simulink library "lib_SecCtrl_MatricesDelayLim"  (R2026a)
settings: Solver=VariableStepAuto
undefined symbols (not defined in the file): A_f_sc, A_P_sc, A_Q_sc, A_v_sc, buses_lf, costs, delayM, Qs_lf, sec_control_structure
libraries: simulink x7, sl_discontinuities x2
settings Model: Creator=atomas  LastModifiedBy=atomas

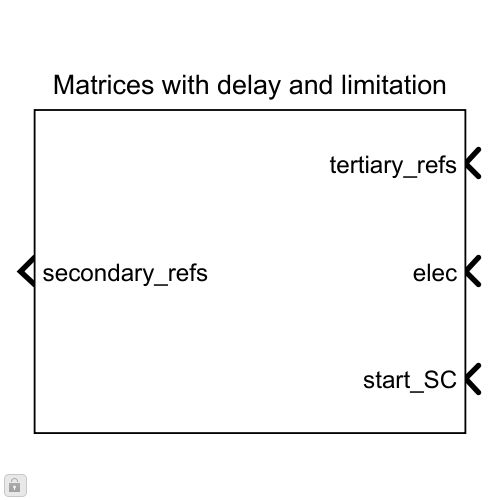
[thumbnail: Simulink's stored preview of the top-level diagram]
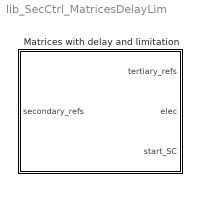
== system lib_SecCtrl_MatricesDelayLim ==
  Matrices with delay and limitation : Subsystem  VariantControl=Matrices with delay and limitation

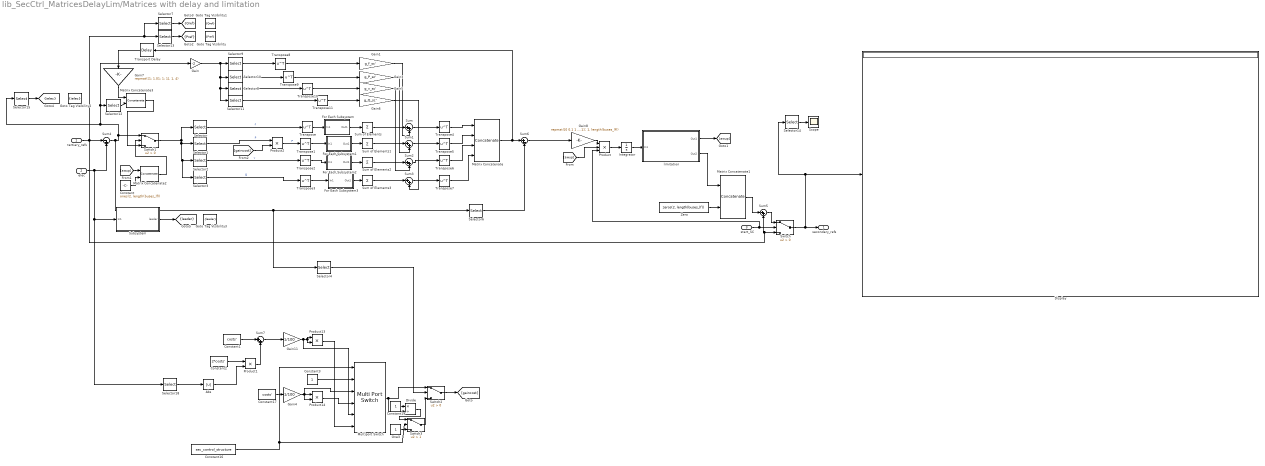
== system lib_SecCtrl_MatricesDelayLim/Matrices with delay and limitation ==
  tertiary_refs : Inport
  elec : Inport  Port=2
  start_SC : Inport  Port=3
  Abs : Abs  SaturateOnIntegerOverflow=off
  Constant : Constant  Value=ones(2, length(buses_lf))  VectorParams1D=off
  Constant1 : Constant  Value=costs'  VectorParams1D=off
  Constant16 : Constant  Value=sec_control_structure
  Constant17 : Constant  Value=costs'  VectorParams1D=off
  Constant19 : Constant  VectorParams1D=off
  Constant2 : Constant  Value=2*costs'  VectorParams1D=off
  Constant3 : Constant
  Display : Display
  Divide : Product  Inputs=*/
  For Each Subsystem : Subsystem  TreatAsAtomicUnit=on  mask{delayM=delayM, A_f_sc=A_f_sc}
  For Each Subsystem1 : Subsystem  TreatAsAtomicUnit=on  mask{delayM=delayM, A_P_sc=A_P_sc}
  For Each Subsystem2 : Subsystem  TreatAsAtomicUnit=on  mask{delayM=delayM, A_v_sc=A_v_sc}
  For Each Subsystem3 : Subsystem  TreatAsAtomicUnit=on  mask{delayM=delayM, A_Q_sc=A_Q_sc}
  Gain : Gain  Gain=-2
  Gain1 : Gain  Gain=g_f_sc'
  Gain11 : Gain  Gain=1/100
  Gain3 : Gain  Gain=g_P_sc'
  Gain4 : Gain  Gain=1/100
  Gain5 : Gain  Gain=g_v_sc'
  Gain6 : Gain  Gain=g_Q_sc'
  Gain7 : Gain  Gain=repmat([1; 1.01; 1; 1], 1, 4)
  Gain8 : Gain  Gain=repmat([0 0.1 1 0.1]', 1, length(buses_lf))
  Goto Tag Visibility : GotoTagVisibility  GotoTag=Pref
  Goto Tag Visibility1 : GotoTagVisibility  GotoTag=Qref
  Goto Tag Visibility2 : GotoTagVisibility  GotoTag=ielec
  Goto Tag Visibility3 : GotoTagVisibility  GotoTag=leader
  Integrator : Integrator
  Matrix Concatenate : Concatenate  NumInputs=4  Mode=Multidimensional array
  Matrix Concatenate1 : Concatenate  Mode=Multidimensional array
  Matrix Concatenate2 : Concatenate  Mode=Multidimensional array
  Matrix Concatenate3 : Concatenate  Mode=Multidimensional array
  Multiport Switch : MultiPortSwitch  Inputs=5  SaturateOnIntegerOverflow=off  InputSameDT=off
  One3 : Constant  OutDataTypeStr=Inherit: Inherit via back propagation
  Product : Product  Inputs=3
  Product{1..2,13..14} (4 alike) : Product
  Scope : Scope
      settings: ActiveDisplayYMinimum=0.00424  ActiveDisplayYMaximum=0.00539
  Selector : Selector  NumberOfDimensions=2  InputPortWidth=3  IndexOptions=Index vector (dialog),Select all  Indices=1,1  OutputSizes=1,1
  Selector{1,4,10,13,18} (5 alike) : Selector  NumberOfDimensions=2  InputPortWidth=3  IndexOptions=Index vector (dialog),Select all  Indices=2,1  OutputSizes=1,1
  Selector11 : Selector  NumberOfDimensions=2  InputPortWidth=3  IndexOptions=Index vector (dialog),Select all  Indices=4,1  OutputSizes=1,1
  Selector12 : Selector  NumberOfDimensions=2  InputPortWidth=3  IndexOptions=Index vector (dialog),Select all  Indices=5:6,1  OutputSizes=1,1
  Selector14 : Selector  NumberOfDimensions=2  InputPortWidth=3  IndexOptions=Index vector (dialog),Index vector (dialog)  Indices=2,1  OutputSizes=1,1
  Selector15 : Selector  NumberOfDimensions=2  InputPortWidth=3  IndexOptions=Index vector (dialog),Select all  Indices=1:4,1  OutputSizes=1,1
  Selector2 : Selector  NumberOfDimensions=2  InputPortWidth=3  IndexOptions=Index vector (dialog),Select all  Indices=3,1  OutputSizes=1,1
  Selector3 : Selector  NumberOfDimensions=2  InputPortWidth=3  IndexOptions=Index vector (dialog),Select all  Indices=4,1  OutputSizes=1,1
  Selector6 : Selector  NumberOfDimensions=2  InputPortWidth=3  IndexOptions=Index vector (dialog),Select all  Indices=1:4,1  OutputSizes=1,1
  Selector7 : Selector  NumberOfDimensions=2  InputPortWidth=3  IndexOptions=Index vector (dialog),Select all  Indices=4,1  OutputSizes=1,1
  Selector8 : Selector  NumberOfDimensions=2  InputPortWidth=3  IndexOptions=Index vector (dialog),Select all  Indices=3,1  OutputSizes=1,1
  Selector9 : Selector  NumberOfDimensions=2  InputPortWidth=3  IndexOptions=Index vector (dialog),Select all  Indices=1,1  OutputSizes=1,1
  Subsystem : Subsystem
  Sum{,1..3,5,7} (6 alike) : Sum  Inputs=|++
  Sum of Elements{,1..3} (4 alike) : Sum  Inputs=+  CollapseMode=Specified dimension  CollapseDim=2
  Sum4 : Sum  Inputs=|-+
  Sum6 : Sum  Inputs=|+-
  Switch : Switch  Criteria=u2 > Threshold  SaturateOnIntegerOverflow=off  InputSameDT=off
  Switch1 : Switch  Criteria=u2 > Threshold  SaturateOnIntegerOverflow=off  InputSameDT=off
  Switch2 : Switch  Criteria=u2 > Threshold  SaturateOnIntegerOverflow=off  InputSameDT=off
  Switch3 : Switch  Criteria=u2 > Threshold  Threshold=1  SaturateOnIntegerOverflow=off  InputSameDT=off
  Transport Delay : TransportDelay  DelayTime=1e-9
  Transpose{,1..11} (12 alike) : Math  Operator=transpose
  Zero : Constant  Value=zeros(2, length(buses_lf))  VectorParams1D=off  OutDataTypeStr=Inherit: Inherit via back propagation
  limitation : Subsystem
  secondary_refs : Outport
  tag scope: Pref=scoped, Qref=scoped, ielec=scoped, leader=scoped
  wires:
  Abs/1 -> Product1/2
  Gain7/1 -> Matrix Concatenate3/1
  Matrix Concatenate3/1 -> Switch1/3
  Selector1/1 -> Product2/1  "P"
  Constant17/1 -> Gain4/1
  Constant19/1 -> Divide/1
  Constant2/1 -> Product1/1
  Product14/1 -> Multiport Switch/4
  Constant3/1 -> Multiport Switch/2
  Switch2/1 -> [gaincost]
  Switch3/1 -> Switch2/3
  Divide/1 -> Switch3/1
  Product13/1 -> Multiport Switch/6
  Product1/1 -> Sum7/2
  Selector18/1 -> Abs/1
  Multiport Switch/1 -> Switch2/1, Divide/2
  Selector4/1 -> Switch2/2
  [gaincost] -> Product2/2
  Constant16/1 -> Multiport Switch/1, Switch3/2
  Constant1/1 -> Sum7/1
  One3/1 -> Switch3/3
  Gain11/1 -> Product13/1, Product13/2, Multiport Switch/5
  Gain4/1 -> Product14/1, Product14/2, Multiport Switch/3
  Sum7/1 -> Gain11/1
  elec/1 -> Sum4/2, Subsystem/1(In1), Selector18/1
  [awup] -> Product/2
  Product/1 -> Integrator/1
  Integrator/1 -> limitation/1(In1)
  Sum6/1 -> Gain8/1
  Zero/1 -> Matrix Concatenate1/2
  tertiary_refs/1 -> Sum4/1, Selector13/1, Selector7/1, Switch/3, Sum5/2
  Selector15/1 -> [ielec]
  Subsystem/1(leader) -> [leader]
  Selector14/1 -> Scope/1
  Transport Delay/1 -> Gain7/1
  Selector12/1 -> Matrix Concatenate3/2
  Sum4/1 -> Selector6/1, Selector4/1, Selector12/1, Gain/1, Selector15/1, Switch1/1
  Constant/1 -> Matrix Concatenate2/2
  [awup] -> Matrix Concatenate2/1
  Matrix Concatenate2/1 -> Switch1/2
  Gain8/1 -> Product/1
  limitation/2(Out2) -> Matrix Concatenate1/1
  limitation/1(Out1) -> [awup]
  Selector7/1 -> [Qref]
  Selector13/1 -> [Pref]
  Gain/1 -> Selector9/1, Selector10/1, Selector8/1, Selector11/1
  Transpose11/1 -> Gain6/1
  Transpose10/1 -> Gain5/1
  Transpose9/1 -> Gain3/1
  Transpose8/1 -> Gain1/1
  start_SC/1 -> Switch/2, Product/3
  Selector6/1 -> Sum6/2
  Matrix Concatenate/1 -> Sum6/1, Transport Delay/1
  Selector9/1 -> Transpose8/1
  Switch1/1 -> Selector/1, Selector1/1, Selector3/1, Selector2/1
  Selector11/1 -> Transpose11/1
  Selector8/1 -> Transpose10/1
  Selector10/1 -> Transpose9/1
  Sum5/1 -> Switch/1
  Matrix Concatenate1/1 -> Sum5/1
  Transpose5/1 -> Matrix Concatenate/2
  Switch/1 -> secondary_refs/1, Display/1, Selector14/1
  For Each Subsystem3/1(Out1) -> Sum of Elements3/1
  For Each Subsystem2/1(Out1) -> Sum of Elements2/1
  For Each Subsystem1/1(Out1) -> Sum of Elements1/1
  For Each Subsystem/1(Out1) -> Sum of Elements/1
  Sum of Elements/1 -> Sum/1
  Transpose7/1 -> Matrix Concatenate/4
  Transpose6/1 -> Matrix Concatenate/3
  Transpose4/1 -> Matrix Concatenate/1
  Transpose3/1 -> For Each Subsystem3/1(In1)
  Transpose2/1 -> For Each Subsystem2/1(In1)
  Transpose1/1 -> For Each Subsystem1/1(In1)
  Transpose/1 -> For Each Subsystem/1(In1)
  Sum of Elements3/1 -> Sum3/1
  Sum3/1 -> Transpose7/1
  Sum2/1 -> Transpose6/1
  Gain6/1 -> Sum3/2
  Gain5/1 -> Sum2/2
  Sum of Elements2/1 -> Sum2/1
  Sum1/1 -> Transpose5/1
  Gain3/1 -> Sum1/2
  Sum of Elements1/1 -> Sum1/1
  Gain1/1 -> Sum/2
  Sum/1 -> Transpose4/1
  Selector2/1 -> Transpose2/1  "v"
  Product2/1 -> Transpose1/1  "P"
  Selector/1 -> Transpose/1  "f"
  Selector3/1 -> Transpose3/1  "Q"

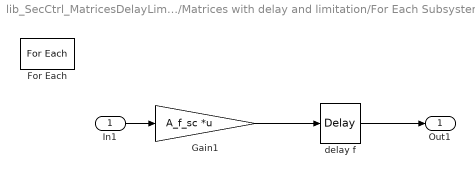
== system lib_SecCtrl_MatricesDelayLim/Matrices with delay and limitation/For Each Subsystem ==
  In1 : Inport  Partition=on  PartitionDimension=1  PartitionWidth=1  PartitionOffset=0
  For Each : ForEach  DisableCoverage=on  IterateSubsysMaskParameter=on,on  SubsysMaskParameterIterationDimension=2,2
  Gain1 : Gain  Gain=A_f_sc  Multiplication=Matrix(K*u)
  delay f : TransportDelay  DelayTime=delayM  PadeOrder=3
  Out1 : Outport  ConcatenationDimension=2
  wires:
  delay f/1 -> Out1/1
  Gain1/1 -> delay f/1
  In1/1 -> Gain1/1

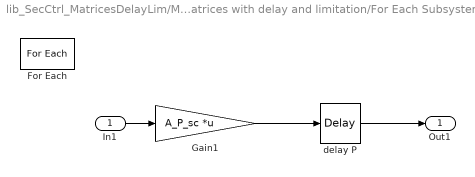
== system lib_SecCtrl_MatricesDelayLim/Matrices with delay and limitation/For Each Subsystem1 ==
  In1 : Inport  Partition=on  PartitionDimension=1  PartitionWidth=1  PartitionOffset=0
  For Each : ForEach  DisableCoverage=on  IterateSubsysMaskParameter=on,on  SubsysMaskParameterIterationDimension=2,2
  Gain1 : Gain  Gain=A_P_sc  Multiplication=Matrix(K*u)
  delay P : TransportDelay  DelayTime=delayM  PadeOrder=3
  Out1 : Outport  ConcatenationDimension=2
  wires:
  In1/1 -> Gain1/1
  Gain1/1 -> delay P/1
  delay P/1 -> Out1/1

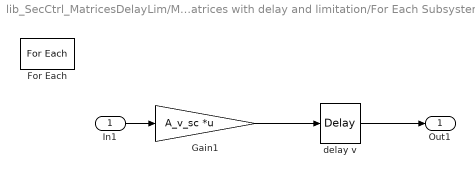
== system lib_SecCtrl_MatricesDelayLim/Matrices with delay and limitation/For Each Subsystem2 ==
  In1 : Inport  Partition=on  PartitionDimension=1  PartitionWidth=1  PartitionOffset=0
  For Each : ForEach  DisableCoverage=on  IterateSubsysMaskParameter=on,on  SubsysMaskParameterIterationDimension=2,2
  Gain1 : Gain  Gain=A_v_sc  Multiplication=Matrix(K*u)
  delay v : TransportDelay  DelayTime=delayM  PadeOrder=3
  Out1 : Outport  ConcatenationDimension=2
  wires:
  delay v/1 -> Out1/1
  Gain1/1 -> delay v/1
  In1/1 -> Gain1/1

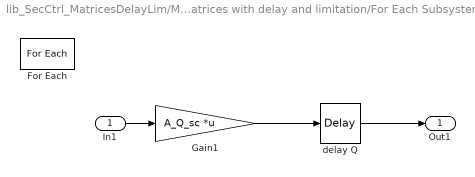
== system lib_SecCtrl_MatricesDelayLim/Matrices with delay and limitation/For Each Subsystem3 ==
  In1 : Inport  Partition=on  PartitionDimension=1  PartitionWidth=1  PartitionOffset=0
  For Each : ForEach  DisableCoverage=on  IterateSubsysMaskParameter=on,on  SubsysMaskParameterIterationDimension=2,2
  Gain1 : Gain  Gain=A_Q_sc  Multiplication=Matrix(K*u)
  delay Q : TransportDelay  DelayTime=delayM  PadeOrder=3
  Out1 : Outport  ConcatenationDimension=2
  wires:
  In1/1 -> Gain1/1
  Gain1/1 -> delay Q/1
  delay Q/1 -> Out1/1

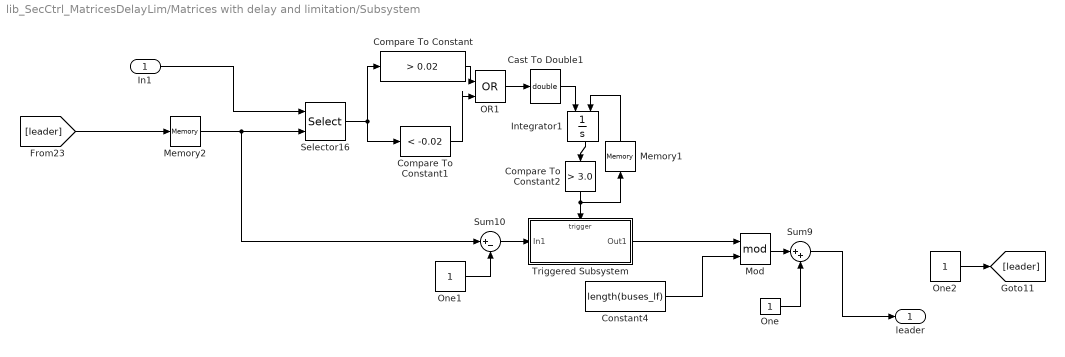
== system lib_SecCtrl_MatricesDelayLim/Matrices with delay and limitation/Subsystem ==
  In1 : Inport
  Cast To Double1 : DataTypeConversion  OutDataTypeStr=double  SaturateOnIntegerOverflow=off  RndMeth=Floor
  Compare To Constant : simulink/Logic and Bit Operations/Compare To Constant  relop=>  const=0.02  OutDataTypeStr=boolean
  Compare To Constant1 : simulink/Logic and Bit Operations/Compare To Constant  relop=<  const=-0.02  OutDataTypeStr=boolean
  Compare To Constant2 : simulink/Logic and Bit Operations/Compare To Constant  relop=>  const=3.0  OutDataTypeStr=boolean
  Constant4 : Constant  Value=length(buses_lf)
  Integrator1 : Integrator  ExternalReset=rising
  Memory1 : Memory
  Memory2 : Memory  InitialCondition=1
  Mod : Math  Operator=mod
  OR1 : Logic  Operator=OR  IconShape=distinctive  AllPortsSameDT=off  OutDataTypeStr=boolean
  One : Constant  OutDataTypeStr=Inherit: Inherit via back propagation
  One1 : Constant  OutDataTypeStr=Inherit: Inherit via back propagation
  One2 : Constant  OutDataTypeStr=Inherit: Inherit via back propagation
  Selector16 : Selector  NumberOfDimensions=2  InputPortWidth=length(buses_lf)  IndexOptions=Index vector (dialog),Index vector (port)  Indices=2,1  OutputSizes=1,1
  Sum10 : Sum  Inputs=|+-
  Sum9 : Sum  Inputs=|++
  Triggered Subsystem : Subsystem  TreatAsAtomicUnit=on
  leader : Outport
  wires:
  One2/1 -> [leader]
  Triggered Subsystem/1(Out1) -> Mod/1
  Memory1/1 -> Integrator1/2
  Sum9/1 -> leader/1
  One1/1 -> Sum10/2
  Constant4/1 -> Mod/2
  Selector16/1 -> Compare To Constant/1, Compare To Constant1/1
  Mod/1 -> Sum9/1
  In1/1 -> Selector16/1
  Sum10/1 -> Triggered Subsystem/1(In1)
  Memory2/1 -> Selector16/2, Sum10/1
  One/1 -> Sum9/2
  Compare To Constant1/1 -> OR1/2
  Cast To Double1/1 -> Integrator1/1
  Integrator1/1 -> Compare To Constant2/1
  OR1/1 -> Cast To Double1/1
  Compare To Constant2/1 -> Triggered Subsystem/Trigger, Memory1/1
  [leader] -> Memory2/1
  Compare To Constant/1 -> OR1/1

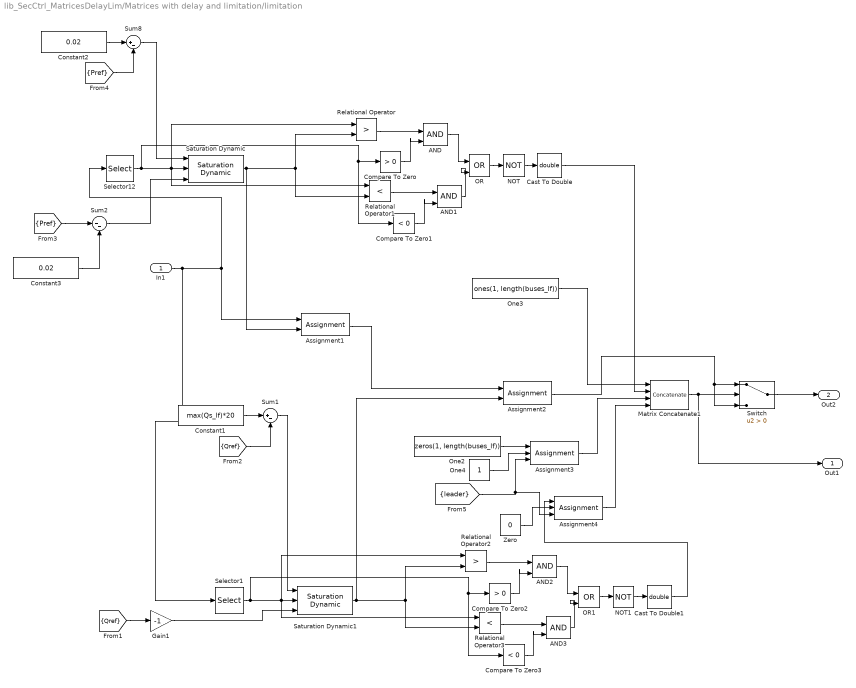
== system lib_SecCtrl_MatricesDelayLim/Matrices with delay and limitation/limitation ==
  In1 : Inport
  AND{,1..3} (4 alike) : Logic  IconShape=distinctive  AllPortsSameDT=off  OutDataTypeStr=boolean
  Assignment1 : Assignment  NumberOfDimensions=2  DiagnosticForDimensions=Warning  IndexOptions=Index vector (dialog),Assign all  Indices=2,1  OutputSizes=1,1
  Assignment2 : Assignment  NumberOfDimensions=2  DiagnosticForDimensions=Warning  IndexOptions=Index vector (dialog),Assign all  Indices=4,1  OutputSizes=1,1
  Assignment3 : Assignment  DiagnosticForDimensions=Warning  IndexOptions=Index vector (port)  Indices=4  OutputSizes=1
  Assignment4 : Assignment  DiagnosticForDimensions=Warning  IndexOptions=Index vector (port)  Indices=4  OutputSizes=1
  Cast To Double : DataTypeConversion  OutDataTypeStr=double  SaturateOnIntegerOverflow=off  RndMeth=Floor
  Cast To Double1 : DataTypeConversion  OutDataTypeStr=double  SaturateOnIntegerOverflow=off  RndMeth=Floor
  Compare To Zero : simulink/Logic and Bit Operations/Compare To Zero  relop=>  OutDataTypeStr=boolean
  Compare To Zero1 : simulink/Logic and Bit Operations/Compare To Zero  relop=<  OutDataTypeStr=boolean
  Compare To Zero2 : simulink/Logic and Bit Operations/Compare To Zero  relop=>  OutDataTypeStr=boolean
  Compare To Zero3 : simulink/Logic and Bit Operations/Compare To Zero  relop=<  OutDataTypeStr=boolean
  Constant1 : Constant  Value=max(Qs_lf)*20  VectorParams1D=off
  Constant2 : Constant  Value=0.02  VectorParams1D=off
  Constant3 : Constant  Value=0.02  VectorParams1D=off
  Gain1 : Gain  Gain=-1
  Matrix Concatenate1 : Concatenate  NumInputs=4  Mode=Multidimensional array
  NOT : Logic  Operator=NOT  IconShape=distinctive  AllPortsSameDT=off  OutDataTypeStr=boolean
  NOT1 : Logic  Operator=NOT  IconShape=distinctive  AllPortsSameDT=off  OutDataTypeStr=boolean
  OR : Logic  Operator=OR  IconShape=distinctive  AllPortsSameDT=off  OutDataTypeStr=boolean
  OR1 : Logic  Operator=OR  IconShape=distinctive  AllPortsSameDT=off  OutDataTypeStr=boolean
  One2 : Constant  Value=zeros(1, length(buses_lf))  VectorParams1D=off  OutDataTypeStr=Inherit: Inherit via back propagation
  One3 : Constant  Value=ones(1, length(buses_lf))  VectorParams1D=off  OutDataTypeStr=Inherit: Inherit via back propagation
  One4 : Constant  OutDataTypeStr=Inherit: Inherit via back propagation
  Relational Operator : RelationalOperator  Operator=>  OutDataTypeStr=boolean  RndMeth=Simplest  InputSameDT=off
  Relational Operator1 : RelationalOperator  Operator=<  OutDataTypeStr=boolean  RndMeth=Simplest  InputSameDT=off
  Relational Operator2 : RelationalOperator  Operator=>  OutDataTypeStr=boolean  RndMeth=Simplest  InputSameDT=off
  Relational Operator3 : RelationalOperator  Operator=<  OutDataTypeStr=boolean  RndMeth=Simplest  InputSameDT=off
  Saturation Dynamic : sl_discontinuities/Saturation Dynamic  OutMin=[]  OutMax=[]  OutDataTypeStr=Inherit: Same as second input  OutDataType=fixdt(1, 16)  OutScaling=2^-10  DoSatur=off
  Saturation Dynamic1 : sl_discontinuities/Saturation Dynamic  OutMin=[]  OutMax=[]  OutDataTypeStr=Inherit: Same as second input  OutDataType=fixdt(1, 16)  OutScaling=2^-10  DoSatur=off
  Selector1 : Selector  NumberOfDimensions=2  InputPortWidth=3  IndexOptions=Index vector (dialog),Select all  Indices=4,1  OutputSizes=1,1
  Selector12 : Selector  NumberOfDimensions=2  InputPortWidth=3  IndexOptions=Index vector (dialog),Select all  Indices=2,1  OutputSizes=1,1
  Sum1 : Sum  Inputs=|+-
  Sum2 : Sum  Inputs=|--
  Sum8 : Sum  Inputs=|+-
  Switch : Switch  Criteria=u2 > Threshold  SaturateOnIntegerOverflow=off  InputSameDT=off
  Zero : Constant  Value=0  OutDataTypeStr=Inherit: Inherit via back propagation
  Out1 : Outport
  Out2 : Outport  Port=2
  wires:
  Constant3/1 -> Sum2/2
  [Pref] -> Sum2/1
  Zero/1 -> Assignment4/2
  Assignment4/1 -> Matrix Concatenate1/4
  One4/1 -> Assignment3/2
  One2/1 -> Assignment3/1
  [leader] -> Assignment3/3, Assignment4/3
  Assignment3/1 -> Matrix Concatenate1/3
  One3/1 -> Matrix Concatenate1/1
  Switch/1 -> Out2/1
  Assignment2/1 -> Switch/1, Switch/3
  Matrix Concatenate1/1 -> Switch/2, Out1/1
  Compare To Zero2/1 -> AND2/2
  Cast To Double1/1 -> Assignment4/1
  In1/1 -> Assignment1/1, Selector12/1, Selector1/1
  [Qref] -> Gain1/1
  Compare To Zero3/1 -> AND3/2
  Sum1/1 -> Saturation Dynamic1/1
  AND2/1 -> OR1/1
  Relational Operator3/1 -> AND3/1
  Selector1/1 -> Compare To Zero2/1, Compare To Zero3/1, Saturation Dynamic1/2, Relational Operator2/1, Relational Operator3/1
  OR1/1 -> NOT1/1
  Gain1/1 -> Saturation Dynamic1/3
  AND3/1 -> OR1/2
  Relational Operator2/1 -> AND2/1
  [Qref] -> Sum1/2
  NOT1/1 -> Cast To Double1/1
  Constant1/1 -> Sum1/1
  Saturation Dynamic1/1 -> Relational Operator2/2, Relational Operator3/2, Assignment2/2
  Assignment1/1 -> Assignment2/1
  Cast To Double/1 -> Matrix Concatenate1/2
  NOT/1 -> Cast To Double/1
  Constant2/1 -> Sum8/1
  Saturation Dynamic/1 -> Relational Operator/2, Relational Operator1/2, Assignment1/2
  Relational Operator/1 -> AND/1
  Sum2/1 -> Saturation Dynamic/3
  OR/1 -> NOT/1
  AND/1 -> OR/1
  AND1/1 -> OR/2
  [Pref] -> Sum8/2
  Sum8/1 -> Saturation Dynamic/1
  Selector12/1 -> Compare To Zero/1, Compare To Zero1/1, Saturation Dynamic/2, Relational Operator/1, Relational Operator1/1
  Compare To Zero1/1 -> AND1/2
  Compare To Zero/1 -> AND/2
  Relational Operator1/1 -> AND1/1

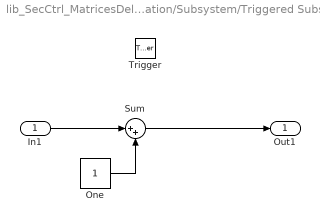
== system lib_SecCtrl_MatricesDelayLim/Matrices with delay and limitation/Subsystem/Triggered Subsystem ==
  In1 : Inport
  Trigger : TriggerPort  VariantControl=(inherit)
  One : Constant  OutDataTypeStr=Inherit: Inherit via back propagation
  Sum : Sum  Inputs=|++
  Out1 : Outport
  wires:
  Sum/1 -> Out1/1
  One/1 -> Sum/2
  In1/1 -> Sum/1
